simulink model "SpeedGoatLoop_v3"  (R2020b)
settings: Solver=FixedStepAuto  StartTime=0.0  StopTime=60*60*1.5  RelTol=1e-3
libraries: fl_lib x42, nesl_utility x19, SimscapeFluids_lib x4, speedgoatlib_IO132 x2, slpidlib x2
(part 1 of 2)
settings Model: SimulationMode=external  EnablePacing=on  PacingRate=100  Creator=cheap  LastModifiedBy=cheap
settings SolverCC: ConcurrentTasks=on  PositivePriorityOrder=on
settings OptimizationCC: BlockReduction=off  OptimizeBlockIOStorage=off
settings DebuggingCC: TasksWithSamePriorityMsg=none
settings HardwareCC: ProdBitPerLong=64  ProdLongLongMode=on  ProdHWDeviceType=Intel->x86-64 (Linux 64)
settings RTWCC: Description=Simulink Real-Time  SystemTargetFile=slrealtime.tlc  TemplateMakefile=slrealtime_default_tmf  Toolchain=Simulink Real-Time Toolchain  BuildConfiguration=Faster Runs  CodeExecutionProfiling=on  TargetLang=C++

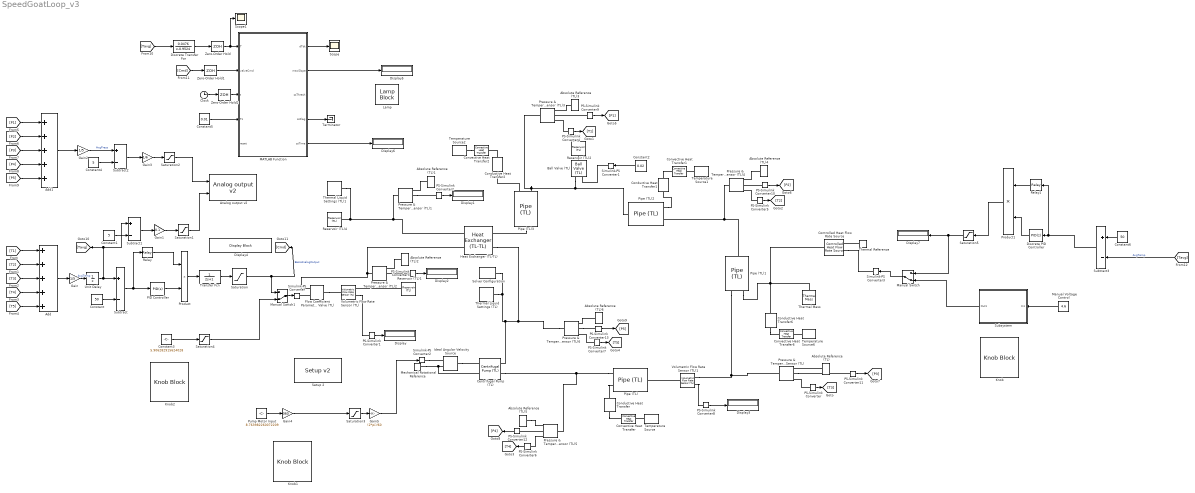
== system SpeedGoatLoop_v3 ==
  Absolute Reference (TL){,1..6} (7 alike) : fl_lib/Thermal Liquid/Elements/Absolute Reference (TL)
      settings: SourceProductBaseCode=SS
  Add : Sum  Inputs=+++++
  Add1 : Sum  Inputs=+++++
  "Analog output v2 " : speedgoatlib_IO132/Analog output v2   parModuleId=1  parSampleTime=-1  parPciSlot=-1  parDacChannels=[1 2]  parDacVoltageRange=[2 2 1 1]  parDacInitValues=[1 1]  parDacReset=[1 1]  parDacSyncOut=1  parDacDmaEnable=0  parDacActiveDmaDevices=1  parDacDmaLatency=2  parDacFrameSize=100
      settings: SourceProductName=Simulink Real-Time: Speedgoat I/O Blockset
  Ball Valve (TL) : SimscapeFluids_lib/Thermal Liquid/Valves & Orifices/Flow Control Valves/Ball Valve (TL)  valve_seat_spec=1  cone_angle=120 deg  diam_ball=1.7 in  diam_orifice=1.5 in  x_0=0 m  area_leak=1e-12 m^2  smoothing_factor=0.05  area=((1.7*pi)^2)/4 in^2  length=0.1 m  Cd=0.7  Re_c=12  mdot_A_specify=off  mdot_A_priority=None  mdot_A=1 kg/s  mdot_A_nominal_specify=off  mdot_A_nominal_unit=kg/s  mdot_A_nominal_value=1
      settings: SourceProductBaseCode=SH  InternalSimscapePortConfiguration="{\"Bottom\":[],\"Left\":[{\"id\":\"A\",\"label\":\"A\",\"type\":\"foundation.thermal_liquid.thermal_liquid\"},{\"id\":\"S\",\"label\":\"S\",\"type\":\"input\"}],\"Right\":[{\"id\":\"B\",\"label\":\"B\",\"type\":\"foundation.thermal_liquid.thermal_liquid\"}],\"Top\":[]}"
  Centrifugal Pump (TL) : SimscapeFluids_lib/Thermal Liquid/Pumps & Motors/Centrifugal Pump (TL)  pump_parameterization=1  mech_orientation=1  flow_rate_1D_TLU=[0 8.33e-5 1.67e-4 2.50e-4 3.33e-4 4.17e-4 5.00e-4 5.83e-4 6.67e-4] m^3/s  head_1D_TLU=[20 19.7 19.0 18.0 16.8 15.2 13.0 10.2 7.5] m  power_1D_TLU=[0 40 80 140 210 290 380 470 550] W  rho_ref_1D=998 kg/m^3  omega_ref_1D=363 rad/s  flow_rate_2D_TLU=[16.67, 23.33, 30, 40, 53.33, 60] lpm  omega_2D_TLU=[2450, 2800, 3150, 3500] rpm  head_2D_TLU=[25, 32.7, 42.5, 50; 24, 31.7, 41, 49; 22.7, 30.5, 39, 47.5; 20, 28, 36, 45; 15.7, 24, 32, 40; 12.5, 21, 29.5, 37.5] m  power_2D_TLU=[.28, .38, .5, .6; .31, .41, .55, .68; .33, .44, .6, .75; .36, .48, .65, .83; .38, .53, .72, .93; .39, .55, .75, .97] kW  rho_ref_2D=920 kg/m^3  omega_threshold=10 rad/s  area=((pi*2)^2)/4 in^2  mdot_A_specify=off  mdot_A_priority=None  mdot_A=1 kg/s  mdot_A_nominal_specify=off  mdot_A_nominal_unit=kg/s  mdot_A_nominal_value=1
      settings: SourceProductBaseCode=SH  InternalSimscapePortConfiguration="{\"Bottom\":[],\"Left\":[{\"id\":\"A\",\"label\":\"A\",\"type\":\"foundation.thermal_liquid.thermal_liquid\"},{\"id\":\"B\",\"label\":\"B\",\"type\":\"foundation.thermal_liquid.thermal_liquid\"}],\"Right\":[{\"id\":\"R\",\"label\":\"R\",\"type\":\"foundation.mechanical.rotational.rotational\"},{\"id\":\"C\",\"label\":\"C\",\"type\":\"foundation.mechanical.rotational.rotational\"}],\"Top\":[]}"
  Clock : Clock
  Conductive Heat Transfer{,1..2,6} (4 alike) : fl_lib/Thermal/Thermal Elements/Conductive Heat Transfer  area=1e-4 m^2  thickness=0.1 m  th_cond=16.2 W/(K*m)  T_specify=off  T_priority=None  T=0 K  T_nominal_specify=off  T_nominal_unit=K  T_nominal_value=1  Q_specify=off  Q_priority=None  Q=0 W  Q_nominal_specify=off  Q_nominal_unit=W  Q_nominal_value=1
  Constant : Constant  Value=50
  Constant1 : Constant  Value=5
  Constant2 : Constant  Value=0.02
  Constant3 : Constant  Value=5.906282915624028
  Constant4 : Constant  Value=5
  Constant5 : Constant  Value=0.01
  Constant6 : Constant  Value=50
  Controlled Heat Flow Rate Source : fl_lib/Thermal/Thermal Sources/Controlled Heat Flow Rate Source
  Convective Heat Transfer : fl_lib/Thermal/Thermal Elements/Convective Heat Transfer  area=pi*50*(656.10+50.8+179.35+254) mm^2  heat_tr_coeff=10 W/(K*m^2)  T_specify=off  T_priority=None  T=0 K  T_nominal_specify=off  T_nominal_unit=K  T_nominal_value=1  Q_specify=off  Q_priority=None  Q=0 W  Q_nominal_specify=off  Q_nominal_unit=W  Q_nominal_value=1
  Convective Heat Transfer1 : fl_lib/Thermal/Thermal Elements/Convective Heat Transfer  area=pi*50*(656.10+50.8+179.35+254) mm^2  heat_tr_coeff=10 W/(K*m^2)  T_specify=off  T_priority=None  T=0 K  T_nominal_specify=off  T_nominal_unit=K  T_nominal_value=1  Q_specify=off  Q_priority=None  Q=0 W  Q_nominal_specify=off  Q_nominal_unit=W  Q_nominal_value=1
  Convective Heat Transfer2 : fl_lib/Thermal/Thermal Elements/Convective Heat Transfer  area=pi*50*(656.10+50.8+179.35+254) mm^2  heat_tr_coeff=10 W/(K*m^2)  T_specify=off  T_priority=None  T=0 K  T_nominal_specify=off  T_nominal_unit=K  T_nominal_value=1  Q_specify=off  Q_priority=None  Q=0 W  Q_nominal_specify=off  Q_nominal_unit=W  Q_nominal_value=1
  Convective Heat Transfer6 : fl_lib/Thermal/Thermal Elements/Convective Heat Transfer  area=pi*50*(6000) mm^2  heat_tr_coeff=10 W/(K*m^2)  T_specify=off  T_priority=None  T=0 K  T_nominal_specify=off  T_nominal_unit=K  T_nominal_value=1  Q_specify=off  Q_priority=None  Q=0 W  Q_nominal_specify=off  Q_nominal_unit=W  Q_nominal_value=1
  Discrete Transfer Fcn : DiscreteTransferFcn  Numerator=[0.0476]  Denominator=[1 -0.9524]  SampleTime=0.01
  Discrete PID Controller : slpidlib/PID Controller  Controller=PID  Form=Parallel  TimeDomain=Discrete-time  UseExternalTs=off  SampleTime=0.01  IntegratorMethod=Forward Euler  FilterMethod=Forward Euler  ControllerParametersSource=internal  P=100  I=1.5  D=0  UseFilter=on  N=100  TunerSelectOption=Transfer Function Based (PID Tuner App)  InitialConditionSource=internal  InitialConditionForIntegrator=0  InitialConditionForFilter=0  DifferentiatorICPrevScaledInput=0  ExternalReset=none  TrackingMode=off  Kt=1  LimitOutput=on  SatLimitsSource=internal  UpperSaturationLimit=10000  LowerSaturationLimit=0  LinearizeAsGain=off  AntiWindupMode=back-calculation  Kb=1  POutMin=[]  POutMax=[]  IOutMin=[]  IOutMax=[]  DOutMin=[]  DOutMax=[]  NOutMin=[]  NOutMax=[]  SumOutMin=[]  SumOutMax=[]  SaturationOutMin=[]  SaturationOutMax=[]  PParamMin=[]  PParamMax=[]  IParamMin=[]  IParamMax=[]  DParamMin=[]  DParamMax=[]  NParamMin=[]  NParamMax=[]  KbParamMin=[]  KbParamMax=[]  KtParamMin=[]  KtParamMax=[]  KbOutMin=[]  KbOutMax=[]  KtOutMin=[]  KtOutMax=[]  IntegratorOutMin=[]  IntegratorOutMax=[]  FilterOutMin=[]  FilterOutMax=[]  SumI1OutMin=[]  SumI1OutMax=[]  SumI2OutMin=[]  SumI2OutMax=[]  SumI3OutMin=[]  SumI3OutMax=[]  SumI4OutMin=[]  SumI4OutMax=[]  SumDOutMin=[]  SumDOutMax=[]  DifferentiatorOutMin=[]  DifferentiatorOutMax=[]  FilterDiffOutCoefMin=[]  FilterDiffOutCoefMax=[]  ReciprocalOutMin=[]  ReciprocalOutMax=[]  SumDenOutMin=[]  SumDenOutMax=[]  SumNumOutMin=[]  SumNumOutMax=[]  DivideOutMin=[]  DivideOutMax=[]  UdiffTsProdOutMin=[]  UdiffTsProdOutMax=[]  NTsProdOutMin=[]  NTsProdOutMax=[]  UintegralTsProdOutMin=[]  UintegralTsProdOutMax=[]  UngainTsProdOutMin=[]  UngainTsProdOutMax=[]  IntegratorContinuousStateAttributes=''  IntegratorStateMustResolveToSignalObject=off  IntegratorRTWStateStorageClass=Auto  FilterContinuousStateAttributes=''  FilterStateMustResolveToSignalObject=off  FilterRTWStateStorageClass=Auto  ParallelPVariant=InternalParameters  IdealPVariant=Disabled  IVariant=InternalParameters  DVariant=InternalParameters  IntegratorVariant=Discrete  SatVariant=Enabled  AWVariant=BackCalculation  PCopyVariant=Disabled  TRVariant=Disabled  FdbkBlocksVariant=Forward  IdealPFdbkVariant=Disabled  SatFdbkVariant=Disabled  DerivativeFilterVariant=ForwardEulerFilter  NVariant=InternalParameters  NCopyVariant=Disabled  FilterICVariant=InternalICsFilter  IntegratorICVariant=InternalICs  ExternalResetVariant=Disabled  TRSumVariant=Passthrough  SumFdbkVariant=Disabled  SumVariant=Sum_PID  TsampFilterVariant=InternalTs  TsampNgainVariant=Passthrough  TsampIntegralVariant=Passthrough  ExternalSaturationOutDataTypeStr=Inherit: Same as second input
  Display{,1..3,5..7} (7 alike) : Display
  Display4 : DisplayBlock  LabelPosition=Hide  Format=short  Transparency=1
  Flow Coefficient Parameterized Valve (TL) : SimscapeFluids_lib/Thermal Liquid/Valves & Orifices/Flow Coefficient Parameterized Valve (TL)  flow_coeff_spec=fluids.thermal_liquid.valves.enum.flow_coeff_spec.cv  Cv_max=1  Cv_min=1e-4  Kv_max=1  Kv_min=1e-4  valve_character=fluids.thermal_liquid.valves.enum.valve_opening_spec.linear  rangeability=50  alpha=2  area=((0.75*pi)^2)/4 in^2  length=3 in  Re_c=12  smoothing_factor=0.02  opening_dynamic=simscape.enum.onoff.off  tau=0.1 s  mdot_A_specify=off  mdot_A_priority=None  mdot_A=1 kg/s  mdot_A_nominal_specify=off  mdot_A_nominal_unit=kg/s  mdot_A_nominal_value=1  area_dynamic_specify=off  area_dynamic_priority=High  area_dynamic=1e-10 m^2  area_dynamic_nominal_specify=off  area_dynamic_nominal_unit=m^2  area_dynamic_nominal_value=1
      settings: SourceProductBaseCode=SH  InternalSimscapePortConfiguration="{\"Bottom\":[],\"Left\":[{\"id\":\"A\",\"label\":\"A\",\"type\":\"foundation.thermal_liquid.thermal_liquid\"},{\"id\":\"L\",\"label\":\"L\",\"type\":\"input\"}],\"Right\":[{\"id\":\"B\",\"label\":\"B\",\"type\":\"foundation.thermal_liquid.thermal_liquid\"}],\"Top\":[]}"
  Gain : Gain  Gain=1/5
  Gain1 : Gain  Gain=0.1
  Gain2 : Gain  Gain=1/5
  Gain3 : Gain  Gain=1/6
  Gain4 : Gain  Gain=360
  Gain5 : Gain  Gain=(2*pi)/60
  Heat Exchanger (TL-TL) : SimscapeFluids_lib/Fluid Network Interfaces/Heat Exchangers/Heat Exchanger (TL-TL)  hex_type=fluids.interfaces.enum.flow_arrangement_spec.shell_tube  cross_type=fluids.interfaces.enum.cross_flow_heat_exchanger_TL_TL_spec.mixed_mixed  shell_num=1  NTU_TLU=[.5, 1, 2, 3, 4, 5]  CR_TLU=[0, .25, .5, .75, 1]  eff_TLU=[.3, .3, .3, .3, .3; .6, .55, .5, .47, .43; .85, .76, .68, .61, .55; .94, .83, .72, .65, .58; .98, .86, .75, .66, .58; .99, .86, .75, .66, .58]  wall_thermal_dynamics=simscape.enum.onoff.on  thermal_mass_wall=447 J/K  R_wall=1.984E-3 K/W  min_flow_area_1=1.16E-3 m^2  Dh_press_1=0.00451 m  liquid_volume_1=3E-3 m^3  Re_lam_1=2000  Re_tur_1=4000  pressure_loss_spec_1=fluids.interfaces.enum.pressure_loss_spec.constant  min_flow_area_2=9.19E-4 m^2  Dh_press_2=0.004572 m  liquid_volume_2=8.41E-4 m^3  Re_lam_2=2000  Re_tur_2=4000  pressure_loss_spec_2=fluids.interfaces.enum.pressure_loss_spec.tube_correlation  pressure_loss_coeff_1=0.1  length_press_1=1 m  length_add_1=0.1 m  roughness_1=15e-6 m  Re_friction_TLU_1=[400, 1000, 1500, 3000, 4000, 6000, 10000, 20000, 40000, 60000, 100000, 100000000]  friction_factor_TLU_1=[.264, .112, .071, .0417, .0387, .0268, .025, .0232, .0226, .022, .0214, .0214]  shape_factor_1=64  Re_Euler_TLU_1=[50, 500, 1000, 2000]  Euler_TLU_1=[4.4505, .6864, .4791, .3755]  pressure_loss_coeff_2=0.1  length_press_2=0.9144 m  length_add_2=0.4 m  roughness_2=15e-6 m  Re_friction_TLU_2=[400, 1000, 1500, 3000, 4000, 6000, 10000, 20000, 40000, 60000, 100000, 100000000]  friction_factor_TLU_2=[.264, .112, .071, .0417, .0387, .0268, .025, .0232, .0226, .022, .0214, .0214]  shape_factor_2=64  Re_Euler_TLU_2=[50, 500, 1000, 2000]  Euler_TLU_2=[4.4505, .6864, .4791, .3755]  heat_transfer_spec_1=fluids.interfaces.enum.heat_transfer_spec.constant  heat_transfer_spec_2=fluids.interfaces.enum.heat_transfer_spec.tube_correlation  heat_coeff_1=100 W/(m^2 * K)  length_heat_1=1 m  Nu_lam_1=3.66  Re_Colburn_TLU_1=[100, 150, 1000]  Colburn_factor_TLU_1=[.019, .013, .002]  Re_Nu_TLU_1=[100, 150, 1000]  Pr_Nu_TLU_1=[1, 10]  Nu_TLU_1=[3.72, 4.21; 3.75, 4.44; 4.21, 7.15]  heat_coeff_2=100 W/(m^2 * K)  length_heat_2=0.9144 m  Nu_lam_2=3.66  Re_Colburn_TLU_2=[100, 150, 1000]  Colburn_factor_TLU_2=[.019, .013, .002]  Re_Nu_TLU_2=[100, 150, 1000]  Pr_Nu_TLU_2=[1, 10]  Nu_TLU_2=[3.72, 4.21; 3.75, 4.44; 4.21, 7.15]  heat_transfer_area_1=1.022 m^2  fouling_factor_1=1e-4 m^2*K/W  min_heat_coeff_1=3000 W/(m^2 * K)  heat_transfer_area_2=0.735 m^2  fouling_factor_2=1e-4 m^2*K/W  min_heat_coeff_2=10000 W/(m^2 * K)  dynamic_compressibility_1=simscape.enum.onoff.on  T0_1=10 degC  p0_1=0.101325 MPa  dynamic_compressibility_2=simscape.enum.onoff.on  T0_2=24 degC  p0_2=0.101325 MPa  mdot1_TLU=[.3, .5, .6, .7, 1, 1.4, 1.9, 2.3] kg/s  mdot2_TLU=[.3, .5, 1, 1.3, 1.7, 2, 2.6, 3.3] kg/s  SD_TLU=[.324, .3533, .404, .4253, .4333, .4373, .4453, .4533; .3813, .424, .496, .5307, .544, .5547, .5693, .5787; .4267, .4827, .5813, .6173, .6413, .6573, .672, .6827; .4613, .528, .64, .6987, .7267, .7467, .7707, .7853; .5533, .6467, .8227, .928, .9853, 1.0187, 1.0653, 1.0973; .58, .688, .8853, 1.0147, 1.08, 1.124, 1.176, 1.2147; .624, .7467, .992, 1.148, 1.244, 1.304, 1.3773, 1.4267; .656, .7907, 1.0667, 1.26, 1.376, 1.452, 1.548, 1.612] kW/K  Q_check=fluids.interfaces.enum.SD_max_check.warning  mdot_dp_TLU_1=[.3, .5, 1, 1.5, 2, 2.5] kg/s  p_diff_TLU_1=[3, 5, 10, 25, 35, 50] * 1e-3 MPa  T_ref_in_1=293.15 K  p_ref_in_1=0.101325 MPa  mdot_threshold_1=1e-3 kg/s  area_1=0.01 m^2  mdot_dp_TLU_2=[.3, .5, 1, 1.5, 2, 2.5] kg/s  p_diff_TLU_2=[3, 5, 10, 25, 35, 50] * 1e-3 MPa  T_ref_in_2=293.15 K  p_ref_in_2=0.101325 MPa  mdot_threshold_2=1e-3 kg/s  area_2=0.01 m^2
      settings: SourceProductBaseCode=SH  InternalSimscapePortConfiguration="{\"Bottom\":[],\"Left\":[{\"id\":\"A1\",\"label\":\"A1\",\"type\":\"foundation.thermal_liquid.thermal_liquid\"},{\"id\":\"B1\",\"label\":\"B1\",\"type\":\"foundation.thermal_liquid.thermal_liquid\"}],\"Right\":[{\"id\":\"A2\",\"label\":\"A2\",\"type\":\"foundation.thermal_liquid.thermal_liquid\"},{\"id\":\"B2\",\"label\":\"B2\",\"type\":\"foundation.thermal_liquid.thermal_liquid\"}],\"Top\":[]}"
  Ideal Angular Velocity Source : fl_lib/Mechanical/Mechanical Sources/Ideal Angular Velocity Source
  Knob : KnobBlock  ScaleMax=20
  Knob1 : KnobBlock  ScaleMax=10
  Knob2 : KnobBlock  ScaleMax=1
  Lamp : LampBlock
  MATLAB Function : MATLAB Function  TreatAsAtomicUnit=on
  Manual Switch : ManualSwitch  CurrentSetting=0
  Manual Switch1 : ManualSwitch  CurrentSetting=0
  Manual Voltage Control : Constant  Value=4.6
  Mechanical Rotational Reference : fl_lib/Mechanical/Rotational Elements/Mechanical Rotational Reference
  PID Controller : slpidlib/PID Controller  Controller=PID  Form=Parallel  TimeDomain=Continuous-time  UseExternalTs=off  SampleTime=-1  IntegratorMethod=Forward Euler  FilterMethod=Forward Euler  ControllerParametersSource=internal  P=0.1  I=1e-5  D=0  UseFilter=on  N=100  TunerSelectOption=Transfer Function Based (PID Tuner App)  InitialConditionSource=internal  InitialConditionForIntegrator=0  InitialConditionForFilter=0  DifferentiatorICPrevScaledInput=0  ExternalReset=none  TrackingMode=off  Kt=1  LimitOutput=on  SatLimitsSource=internal  UpperSaturationLimit=1  LowerSaturationLimit=0  LinearizeAsGain=on  AntiWindupMode=clamping  Kb=1  POutMin=[]  POutMax=[]  IOutMin=[]  IOutMax=[]  DOutMin=[]  DOutMax=[]  NOutMin=[]  NOutMax=[]  SumOutMin=[]  SumOutMax=[]  SaturationOutMin=[]  SaturationOutMax=[]  PParamMin=[]  PParamMax=[]  IParamMin=[]  IParamMax=[]  DParamMin=[]  DParamMax=[]  NParamMin=[]  NParamMax=[]  KbParamMin=[]  KbParamMax=[]  KtParamMin=[]  KtParamMax=[]  KbOutMin=[]  KbOutMax=[]  KtOutMin=[]  KtOutMax=[]  IntegratorOutMin=[]  IntegratorOutMax=[]  FilterOutMin=[]  FilterOutMax=[]  SumI1OutMin=[]  SumI1OutMax=[]  SumI2OutMin=[]  SumI2OutMax=[]  SumI3OutMin=[]  SumI3OutMax=[]  SumI4OutMin=[]  SumI4OutMax=[]  SumDOutMin=[]  SumDOutMax=[]  DifferentiatorOutMin=[]  DifferentiatorOutMax=[]  FilterDiffOutCoefMin=[]  FilterDiffOutCoefMax=[]  ReciprocalOutMin=[]  ReciprocalOutMax=[]  SumDenOutMin=[]  SumDenOutMax=[]  SumNumOutMin=[]  SumNumOutMax=[]  DivideOutMin=[]  DivideOutMax=[]  UdiffTsProdOutMin=[]  UdiffTsProdOutMax=[]  NTsProdOutMin=[]  NTsProdOutMax=[]  UintegralTsProdOutMin=[]  UintegralTsProdOutMax=[]  UngainTsProdOutMin=[]  UngainTsProdOutMax=[]  IntegratorContinuousStateAttributes=''  IntegratorStateMustResolveToSignalObject=off  IntegratorRTWStateStorageClass=Auto  FilterContinuousStateAttributes=''  FilterStateMustResolveToSignalObject=off  FilterRTWStateStorageClass=Auto  ParallelPVariant=InternalParameters  IdealPVariant=Disabled  IVariant=InternalParameters  DVariant=InternalParameters  IntegratorVariant=Continuous  SatVariant=Enabled  AWVariant=ContClampingParallel  PCopyVariant=Disabled  TRVariant=Disabled  FdbkBlocksVariant=Forward  IdealPFdbkVariant=Disabled  SatFdbkVariant=Disabled  DerivativeFilterVariant=ContFilter  NVariant=InternalParameters  NCopyVariant=Disabled  FilterICVariant=InternalICsFilter  IntegratorICVariant=InternalICs  ExternalResetVariant=Disabled  TRSumVariant=Passthrough  SumFdbkVariant=Disabled  SumVariant=Sum_PID  TsampFilterVariant=InternalTs  TsampNgainVariant=Passthrough  TsampIntegralVariant=Passthrough  ExternalSaturationOutDataTypeStr=Inherit: Same as second input
  PS-Simulink Converter{,4..7} (5 alike) : nesl_utility/PS-Simulink Converter  PhysicalDomain=network_engine_domain  SubClassName=ps_output  LeftPortType=input  RightPortType=output  PseudoPeriodic=off  Frequencies=[]  Unit=degC  AffineConversion=on
  PS-Simulink Converter1 : nesl_utility/PS-Simulink Converter  PhysicalDomain=network_engine_domain  SubClassName=ps_output  LeftPortType=input  RightPortType=output  PseudoPeriodic=off  Frequencies=[]  Unit=gpm  AffineConversion=on
  PS-Simulink Converter{2,9..13} (6 alike) : nesl_utility/PS-Simulink Converter  PhysicalDomain=network_engine_domain  SubClassName=ps_output  LeftPortType=input  RightPortType=output  PseudoPeriodic=off  Frequencies=[]  Unit=psi  AffineConversion=on
  PS-Simulink Converter3 : nesl_utility/PS-Simulink Converter  PhysicalDomain=network_engine_domain  SubClassName=ps_output  LeftPortType=input  RightPortType=output  PseudoPeriodic=off  Frequencies=[]  Unit=inherit  AffineConversion=off
  PS-Simulink Converter8 : nesl_utility/PS-Simulink Converter  PhysicalDomain=network_engine_domain  SubClassName=ps_output  LeftPortType=input  RightPortType=output  PseudoPeriodic=off  Frequencies=[]  Unit=gpm  AffineConversion=on
  Pipe (TL) : fl_lib/Thermal Liquid/Elements/Pipe (TL)  length=572+698.5+113+656.1+50.8+179.35+254 mm  area=((1.7*pi)^2)/4 in^2  Dh=1.5 in  length_add=1 m  roughness=15e-6 m  Re_lam=2000  Re_tur=4000  shape_factor=64  Nu_lam=3.66  dynamic_compressibility=simscape.enum.onoff.on  inertia=simscape.enum.onoff.off  p0=40 psi  T0=24 degC  mdot0=0 kg/s
      settings: SourceProductBaseCode=SS
  Pipe (TL)1 : fl_lib/Thermal Liquid/Elements/Pipe (TL)  length=1666.08+113 mm  area=((50*pi)^2)/4 mm^2  Dh=1.5 in  length_add=1 m  roughness=15e-6 m  Re_lam=2000  Re_tur=4000  shape_factor=64  Nu_lam=3.66  dynamic_compressibility=simscape.enum.onoff.on  inertia=simscape.enum.onoff.off  p0=0.12 MPa  T0=24 degC  mdot0=0 kg/s
      settings: SourceProductBaseCode=SS
  Pipe (TL)2 : fl_lib/Thermal Liquid/Elements/Pipe (TL)  length=322.66+283.65+665.16+113+331.45+863.6 mm  area=((1.7*pi)^2)/4 in^2  Dh=1.5 in  length_add=1 m  roughness=15e-6 m  Re_lam=2000  Re_tur=4000  shape_factor=64  Nu_lam=3.66  dynamic_compressibility=simscape.enum.onoff.on  inertia=simscape.enum.onoff.off  p0=0.101325 MPa  T0=24 degC  mdot0=0 kg/s
      settings: SourceProductBaseCode=SS
  Pipe (TL)3 : fl_lib/Thermal Liquid/Elements/Pipe (TL)  length=211.02+1024.8+164.52+317.72 mm  area=((1.7*pi)^2)/4 in^2  Dh=1.5 in  length_add=1 m  roughness=15e-6 m  Re_lam=2000  Re_tur=4000  shape_factor=64  Nu_lam=3.66  dynamic_compressibility=simscape.enum.onoff.on  inertia=simscape.enum.onoff.off  p0=0.101325 MPa  T0=24 degC  mdot0=0 kg/s
      settings: SourceProductBaseCode=SS
  Pressure & Temperature Sensor (TL){,1..6} (7 alike) : fl_lib/Thermal Liquid/Sensors/Pressure & Temperature Sensor (TL)
      settings: SourceProductBaseCode=SS  InternalSimscapePortConfiguration="{\"Bottom\":[],\"Left\":[{\"id\":\"A\",\"label\":\"A\",\"type\":\"foundation.thermal_liquid.thermal_liquid\"}],\"Right\":[{\"id\":\"B\",\"label\":\"B\",\"type\":\"foundation.thermal_liquid.thermal_liquid\"},{\"id\":\"P\",\"label\":\"P\",\"type\":\"output\"},{\"id\":\"T\",\"label\":\"T\",\"type\":\"output\"}],\"Top\":[]}"
  Product : Product
  Product1 : Product
  Pump Motor Input : Constant  Value=8.763982260072209
  Relay : Relay  OnSwitchValue=48  OffSwitchValue=46
  Relay1 : Relay  OnSwitchValue=48  OffSwitchValue=46  OnOutputValue=0  OffOutputValue=1
  Reservoir (TL)1 : fl_lib/Thermal Liquid/Elements/Reservoir (TL)  pressure_spec=foundation.enum.pressure_spec.atmospheric  reservoir_pressure=0.101325 MPa  reservoir_temperature=10 degC  area=((pi*1.5)^2)/4 in^2
      settings: SourceProductBaseCode=SS
  Reservoir (TL)2 : fl_lib/Thermal Liquid/Elements/Reservoir (TL)  pressure_spec=foundation.enum.pressure_spec.atmospheric  reservoir_pressure=0.101325 MPa  reservoir_temperature=15 degC  area=((pi*1.5)^2)/4 in^2
      settings: SourceProductBaseCode=SS
  Reservoir (TL)4 : fl_lib/Thermal Liquid/Elements/Reservoir (TL)  pressure_spec=foundation.enum.pressure_spec.specified  reservoir_pressure=60 psi  reservoir_temperature=10 degC  area=((pi*1.5)^2)/4 in^2
      settings: SourceProductBaseCode=SS
  Saturation : Saturate  UpperLimit=0.98  LowerLimit=0.0002
  Saturation1 : Saturate  UpperLimit=10  LowerLimit=0
  Saturation2 : Saturate  UpperLimit=90  LowerLimit=20
  Saturation3 : Saturate  UpperLimit=3600  LowerLimit=0
  Saturation4 : Saturate  LowerLimit=7e-5
  Saturation5 : Saturate  UpperLimit=10000  LowerLimit=0
  Scope : Scope
  Scope1 : Scope
  "Setup 2 " : speedgoatlib_IO132/Setup v2   parPciSlot=-1  parModuleId=1  parInterModuleSync=None  parConvClockBaseRate=20MHz  parConvClock1Divider=20000  parConvClock2Divider=20000  parFrameTriggerEnable=off  parFrameTriggerDivider=10  parConvClock1BaseRate=1  parConvClock2BaseRate=1  parFrameTriggerClock=1  parAdcChannels=[1]  parAdcRange1=+-10V  parAdcOversampling1=None  parAdcAutoCorrection=on  parAdcContSampling=off  parAdcVoltageRange=2  parAdcOversamplRate=1  parAdcDmaEnable=off  parAdcDmaClock=Clock 1  parAdcFrameSize_=100  parAdcSampleTime_=-1  parAdcActiveDmaDevices=[1]  parAdcFrameTriggerEnable=0  parAdcFrameSize=100  parAdcSampleTime=0.1  parDacChannels=[1 2]  parDacInitValues=1  parDacReset=1  parDacRange1=0-10V  parDacRange2=0-10V  parDacRange3=0-5V  parDacRange4=0-5V  parDacVoltageRange=[2 2 1 1]  parDacAutoCorrection=on  parDacSyncOut=on  parDacDmaEnable=off  parDacDmaLatency=Until next frame  parDacDmaClock=Clock 1  parDacFrameSize_=100  parDacSampleTime_=-1  parDacActiveDmaDevices=[1]  parDacFrameTriggerEnable=0  parDacFrameSize=100  parDacSampleTime=0.1  parDoChannels=[1 2]  parDoInitValues=0  parDoReset=1  parDiChannels=[3 4]  parDiDebounceEnable=off  parDiDebounceTime=0  parDiDebounceValue=0  parDioPullRefFront=Pull-up 3.3V  parDioPullRefRear=Floating
      settings: SourceProductName=Simulink Real-Time: Speedgoat Library
  Simulink-PS Converter{,1..3} (4 alike) : nesl_utility/Simulink-PS Converter  PhysicalDomain=network_engine_domain  SubClassName=ps_input  LeftPortType=input  RightPortType=output  PseudoPeriodic=off  Frequencies=[]  NoiseDistribution=none  NoiseParameters=[]  Unit=1  AffineConversion=off  FilteringAndDerivatives=provide  SimscapeFilterOrder=1  InputFilterTimeConstant=0.001  UdotUserProvided=0
  Solver Configuration : nesl_utility/Solver Configuration  PhysicalDomain=network_engine_domain  SubClassName=solver  LeftPortType=input  RightPortType=generic  Tones=[]  Harmonics=[]  SimulateNoise=off  Profile=off  UseLocalSampling=off  EnableSwitchedLinearOptims=on  FrequencyDomain=off  UseCCode=off  RelTol=0.001  AbsTol=1e-06  MinStep=1e-09  ToWorkspace=off  RevertToSquareIcSolve=off  NumHomotopyIterations=100  PhasorMode=off  PhasorModeNumHarmonics=1  DoDC=off  ResidualTolerance=1e-09  UseLocalSolver=on  LocalSolverChoice=NE_BACKWARD_EULER_ADVANCER  LocalSolverSampleTime=0.01  DoFixedCost=on  MaxNonlinIter=3  MaxModeIter=2  ComputeImpulses=off  ImpulseIterations=2  LinearAlgebra=auto  EquationFormulation=NE_TIME_EF  DelaysMemoryBudget=1024  AutomaticFiltering=on  FilteringTimeConstant=0.001  PartitionStorageMethod=AS_NEEDED  PartitionMemoryBudget=1024  PartitionMethod=ROBUST
  Subsystem : Subsystem
      settings: PortSchema="{\"entries\":[{\"content\":{\"sides\":[{\"content\":{\"connectorIds\":[\"Out1\"]},\"type\":\"ConnectorPlacement.EquallySpacedRectSide\",\"uuid\":\"fb919825-1b2f-4c31-9805-0967e26cfa90\"},{\"content\":{\"connectorIds\":[\"In1\"],\"side\":\"RIGHT\"},\"type\":\"ConnectorPlacement.EquallySpacedRectSide\",\"uuid\":\"9136b45b-edcb-43b5-a0c1-cf6d919585f5\"},{\"content\":{\"connectorIds\":[],\"side\":\"TOP\"},\"type\":\"ConnectorPlacement.EquallySpacedRectSide\",\"uuid\":\"eaf0a6cf-ad87-41c1-a56b-7e33ba526407\"}]},\"type\":\"ConnectorPlacement.EquallySpacedConnector\",\"uuid\":\"77377397-7f65-431b-b464-9c22985d1642\"}],\"packageUris\":[\"http://schema.mathworks.com/mf0/Connector/R2020b\"],\"version\":\"1.0\"}"
  Subtract{,1..3} (4 alike) : Sum  Inputs=+-
  Temperature Source{,1..2,6} (4 alike) : fl_lib/Thermal/Thermal Sources/Temperature Source  temperature=293.15 K
  Terminator : Terminator
  Thermal Liquid Settings (TL) : fl_lib/Thermal Liquid/Utilities/Thermal Liquid Settings (TL)  table_dimensions=foundation.enum.table_dimensions_TL.two_dimensional  T_TLU=[5 : 10 : 105]' degC  p_TLU=[0.01, 0.1, 5 : 5 : 50] MPa  p_atm=0.101325 MPa  pT_region_flag=foundation.enum.pT_region_TL.min_max  T_min=5 degC  T_max=105 degC  p_min=0.05 MPa  p_max=50 MPa  T_min_1D=273.16 K  T_max_1D=363.16 K  p_min_1D=0.05 MPa  p_max_1D=50 MPa  pT_validity_TLU=[1, 1, 1, 1, 1, 1, 1, 1, 1, 1, 1, 1; 1, 1, 1, 1, 1, 1, 1, 1, 1, 1, 1, 1; 1, 1, 1, 1, 1, 1, 1, 1, 1, 1, 1, 1; 1, 1, 1, 1, 1, 1, 1, 1, 1, 1, 1, 1; 1, 1, 1, 1, 1, 1, 1, 1, 1, 1, 1, 1; 0, 1, 1, 1, 1, 1, 1, 1, 1, 1, 1, 1; 0, 1, 1, 1, 1, 1, 1, 1, 1, 1, 1, 1; 0, 1, 1, 1, 1, 1, 1, 1, 1, 1, 1, 1; 0, 1, 1, 1, 1, 1, 1, 1, 1, 1, 1, 1; 0, 1, 1, 1, 1, 1, 1, 1, 1, 1, 1, 1; 0, 0, 1, 1, 1, 1, 1, 1, 1, 1, 1, 1]  rho_parameterization_2D=foundation.enum.rho_parameterization_2D.rho_beta_alpha  rho_parameterization_1D=foundation.enum.rho_parameterization_1D.rho_vector  rho_TLU=[999.7973, 999.8431, 1002.3216, 1004.8218, 1007.293, 1009.7358, 1012.1506, 1014.5379, 1016.8979, 1019.2311, 1021.538, 1023.8188; 999.6579, 999.7009, 1002.0303, 1004.382, 1006.7084, 1009.0101, 1011.2874, 1013.5407, 1015.7703, 1017.9766, 1020.1599, 1022.3206; 998.1632, 998.2045, 1000.4375, 1002.6924, 1004.9239, 1007.1324, 1009.3183, 1011.4819, 1013.6236, 1015.7438, 1017.8428, 1019.921; 995.6057, 995.6458, 997.81864, 1000.0128, 1002.1841, 1004.3332, 1006.4603, 1008.566, 1010.6505, 1012.7144, 1014.758, 1016.7815; 992.1724, 992.2119, 994.35133, 996.5113, 998.6484, 1000.7633, 1002.8563, 1004.928, 1006.9788, 1009.009, 1011.0192, 1013.0097; 988.02, 988.0299, 990.15684, 992.3035, 994.4268, 996.5273, 998.6056, 1000.6622, 1002.6976, 1004.7123, 1006.7067, 1008.6813; 983.18, 983.1901, 985.3217, 987.4721, 989.5983, 991.7008, 993.7803, 995.8374, 997.8726, 999.8864, 1001.8795, 1003.8522; 977.75, 977.7583, 979.9094, 982.0783, 984.2216, 986.34, 988.4343, 990.505, 992.5529, 994.5786, 996.5825, 998.5654; 971.77, 971.7836, 973.96734, 976.1678, 978.3409, 980.4876, 982.6087, 984.7049, 986.7768, 988.8254, 990.8511, 992.8545; 965.26, 965.3023, 967.53107, 969.7753, 971.9901, 974.1764, 976.3354, 978.4676, 980.5741, 982.6556, 984.7129, 986.7465; 958.62, 958.6315, 960.627, 962.9267, 965.1944, 967.4314, 969.6387, 971.8173, 973.9681, 976.0921, 978.19, 980.2628] kg/m^3  beta_TLU=[1.9649, 1.9654, 1.9929, 2.0213, 2.0499, 2.0787, 2.1078, 2.1372, 2.1668, 2.1966, 2.2268, 2.2572; 2.0913, 2.0918, 2.1191, 2.1471, 2.1752, 2.2036, 2.2322, 2.261, 2.2899, 2.3191, 2.3485, 2.3781; 2.1786, 2.1791, 2.2067, 2.235, 2.2634, 2.2919, 2.3206, 2.3494, 2.3784, 2.4075, 2.4367, 2.4661; 2.2332, 2.2337, 2.2619, 2.2908, 2.3197, 2.3487, 2.3778, 2.407, 2.4363, 2.4657, 2.4951, 2.5246; 2.26, 2.2605, 2.2895, 2.3191, 2.3487, 2.3784, 2.4081, 2.4378, 2.4675, 2.4973, 2.5272, 2.5571; 2.2638, 2.2638, 2.2936, 2.324, 2.3544, 2.3848, 2.4151, 2.4455, 2.4758, 2.5062, 2.5365, 2.5669; 2.2472, 2.2472, 2.2779, 2.3092, 2.3403, 2.3715, 2.4025, 2.4336, 2.4646, 2.4955, 2.5264, 2.5573; 2.214, 2.214, 2.2455, 2.2776, 2.3096, 2.3415, 2.3733, 2.405, 2.4367, 2.4683, 2.4998, 2.5313; 2.1668, 2.1668, 2.1992, 2.2321, 2.2649, 2.2976, 2.3301, 2.3626, 2.3949, 2.4272, 2.4593, 2.4914; 2.1081, 2.1081, 2.1413, 2.175, 2.2086, 2.2421, 2.2754, 2.3085, 2.3415, 2.3744, 2.4072, 2.4399; 2.0494, 2.0494, 2.0739, 2.1084, 2.1428, 2.177, 2.211, 2.2449, 2.2786, 2.3121, 2.3455, 2.3788] GPa  alpha_TLU=1e-4 * [-.679, -.676, -.49, -.307, -.13, .041, .206, .365, .519, .668, .811, .949; .878, .881, .998, 1.114, 1.227, 1.337, 1.445, 1.549, 1.651, 1.75, 1.846, 1.939; 2.068, 2.069, 2.141, 2.213, 2.283, 2.352, 2.42, 2.486, 2.551, 2.614, 2.676, 2.736; 3.034, 3.035, 3.074, 3.113, 3.152, 3.191, 3.229, 3.267, 3.305, 3.341, 3.377, 3.413; 3.855, 3.856, 3.87, 3.884, 3.899, 3.914, 3.93, 3.946, 3.961, 3.977, 3.993, 4.009; 4.578, 4.578, 4.572, 4.566, 4.562, 4.558, 4.555, 4.552, 4.55, 4.549, 4.548, 4.547; 5.233, 5.233, 5.209, 5.186, 5.165, 5.144, 5.125, 5.107, 5.09, 5.074, 5.059, 5.045; 5.84, 5.84, 5.801, 5.762, 5.725, 5.691, 5.657, 5.625, 5.595, 5.566, 5.538, 5.512; 6.414, 6.414, 6.36, 6.307, 6.256, 6.208, 6.161, 6.117, 6.074, 6.033, 5.994, 5.956; 6.967, 6.967, 6.898, 6.831, 6.766, 6.705, 6.646, 6.589, 6.535, 6.482, 6.432, 6.384; 7.519, 7.519, 7.423, 7.342, 7.264, 7.189, 7.118, 7.049, 6.983, 6.92, 6.859, 6.8] 1/K  rho_TLU_2=[999.7973, 999.8431, 1002.3216, 1004.8218, 1007.293, 1009.7358, 1012.1506, 1014.5379, 1016.8979, 1019.2311, 1021.538, 1023.8188; 999.6579, 999.7009, 1002.0303, 1004.382, 1006.7084, 1009.0101, 1011.2874, 1013.5407, 1015.7703, 1017.9766, 1020.1599, 1022.3206; 998.1632, 998.2045, 1000.4375, 1002.6924, 1004.9239, 1007.1324, 1009.3183, 1011.4819, 1013.6236, 1015.7438, 1017.8428, 1019.921; 995.6057, 995.6458, 997.81864, 1000.0128, 1002.1841, 1004.3332, 1006.4603, 1008.566, 1010.6505, 1012.7144, 1014.758, 1016.7815; 992.1724, 992.2119, 994.35133, 996.5113, 998.6484, 1000.7633, 1002.8563, 1004.928, 1006.9788, 1009.009, 1011.0192, 1013.0097; 988.02, 988.0299, 990.15684, 992.3035, 994.4268, 996.5273, 998.6056, 1000.6622, 1002.6976, 1004.7123, 1006.7067, 1008.6813; 983.18, 983.1901, 985.3217, 987.4721, 989.5983, 991.7008, 993.7803, 995.8374, 997.8726, 999.8864, 1001.8795, 1003.8522; 977.75, 977.7583, 979.9094, 982.0783, 984.2216, 986.34, 988.4343, 990.505, 992.5529, 994.5786, 996.5825, 998.5654; 971.77, 971.7836, 973.96734, 976.1678, 978.3409, 980.4876, 982.6087, 984.7049, 986.7768, 988.8254, 990.8511, 992.8545; 965.26, 965.3023, 967.53107, 969.7753, 971.9901, 974.1764, 976.3354, 978.4676, 980.5741, 982.6556, 984.7129, 986.7465; 958.62, 958.6315, 960.627, 962.9267, 965.1944, 967.4314, 969.6387, 971.8173, 973.9681, 976.0921, 978.19, 980.2628] kg/m^3  rho_ref_3=998.21 kg/m^3  T_ref_3=293.16 K  p_ref_3=0.101325 MPa  beta_const_3=2.1791 GPa  alpha_const_3=2.0691e-4 1/K  rho_TLU_4=[999.84; 999.7; 998.2; 995.65; 992.21; 988.03; 983.19; 977.76; 971.78; 965.3; 958.8] kg/m^3  beta_const_4=2.1791 GPa  p_ref_4=0.101325 MPa  rho_ref_5=998.21 kg/m^3  T_ref_5=293.16 K  p_ref_5=0.101325 MPa  beta_const_5=2.1791 GPa  alpha_const_5=2.0691e-4 1/K  u_parameterization_2D=foundation.enum.u_parameterization_2D.u_cp  u_parameterization_1D=foundation.enum.u_parameterization_1D.u  u_TLU=[.0002, .0018, .086, .1588, .219, .267, .3034, .3288, .3436, .3483, .3435, .3294; 42.062, 42.06, 41.935, 41.804, 41.668, 41.527, 41.382, 41.233, 41.081, 40.924, 40.763, 40.599; 83.953, 83.948, 83.651, 83.349, 83.049, 82.749, 82.451, 82.153, 81.856, 81.56, 81.265, 80.971; 125.77, 125.76, 125.31, 124.86, 124.41, 123.97, 123.53, 123.1, 122.68, 122.25, 121.84, 121.42; 167.57, 167.56, 166.96, 166.37, 165.79, 165.21, 164.65, 164.09, 163.54, 163, 162.46, 161.94; 209.36, 209.36, 208.63, 207.9, 207.19, 206.48, 205.79, 205.11, 204.45, 203.79, 203.14, 202.5; 251.19, 251.19, 250.33, 249.47, 248.62, 247.79, 246.98, 246.18, 245.39, 244.62, 243.86, 243.12; 293.06, 293.06, 292.07, 291.07, 290.1, 289.14, 288.2, 287.28, 286.38, 285.49, 284.62, 283.77; 334.99, 334.99, 333.86, 332.73, 331.63, 330.54, 329.48, 328.44, 327.41, 326.41, 325.43, 324.46; 377, 377, 375.73, 374.46, 373.22, 372, 370.81, 369.64, 368.5, 367.38, 366.27, 365.19; 419.01, 419.01, 417.69, 416.27, 414.89, 413.54, 412.21, 410.91, 409.64, 408.4, 407.17, 405.98] kJ/kg  cp_TLU=[4.2199, 4.2194, 4.1957, 4.1726, 4.1508, 4.13, 4.1103, 4.0916, 4.0738, 4.0569, 4.0408, 4.0254; 4.1955, 4.1951, 4.1769, 4.1592, 4.1422, 4.1259, 4.1103, 4.0954, 4.0812, 4.0676, 4.0545, 4.0421; 4.1843, 4.184, 4.169, 4.1543, 4.1401, 4.1264, 4.1133, 4.1007, 4.0885, 4.0768, 4.0656, 4.0548; 4.1801, 4.1798, 4.1667, 4.1538, 4.1413, 4.1293, 4.1177, 4.1064, 4.0956, 4.0851, 4.075, 4.0653; 4.1796, 4.1794, 4.1675, 4.1558, 4.1444, 4.1334, 4.1227, 4.1123, 4.1023, 4.0926, 4.0832, 4.0741; 4.1813, 4.1813, 4.1702, 4.1592, 4.1484, 4.138, 4.1279, 4.1181, 4.1086, 4.0993, 4.0903, 4.0816; 4.185, 4.185, 4.1742, 4.1636, 4.1532, 4.1432, 4.1334, 4.1239, 4.1146, 4.1056, 4.0969, 4.0884; 4.1901, 4.1901, 4.1795, 4.169, 4.1588, 4.1489, 4.1393, 4.1299, 4.1207, 4.1118, 4.1032, 4.0947; 4.1968, 4.1968, 4.1862, 4.1757, 4.1655, 4.1555, 4.1458, 4.1364, 4.1273, 4.1183, 4.1096, 4.1012; 4.2052, 4.2052, 4.1944, 4.1837, 4.1733, 4.1632, 4.1534, 4.1438, 4.1345, 4.1255, 4.1166, 4.108; 4.2136, 4.2136, 4.2045, 4.1935, 4.1828, 4.1724, 4.1623, 4.1524, 4.1429, 4.1335, 4.1245, 4.1157] kJ/kg/K  u_TLU_2=[.0002, .0018, .086, .1588, .219, .267, .3034, .3288, .3436, .3483, .3435, .3294; 42.062, 42.06, 41.935, 41.804, 41.668, 41.527, 41.382, 41.233, 41.081, 40.924, 40.763, 40.599; 83.953, 83.948, 83.651, 83.349, 83.049, 82.749, 82.451, 82.153, 81.856, 81.56, 81.265, 80.971; 125.77, 125.76, 125.31, 124.86, 124.41, 123.97, 123.53, 123.1, 122.68, 122.25, 121.84, 121.42; 167.57, 167.56, 166.96, 166.37, 165.79, 165.21, 164.65, 164.09, 163.54, 163, 162.46, 161.94; 209.36, 209.36, 208.63, 207.9, 207.19, 206.48, 205.79, 205.11, 204.45, 203.79, 203.14, 202.5; 251.19, 251.19, 250.33, 249.47, 248.62, 247.79, 246.98, 246.18, 245.39, 244.62, 243.86, 243.12; 293.06, 293.06, 292.07, 291.07, 290.1, 289.14, 288.2, 287.28, 286.38, 285.49, 284.62, 283.77; 334.99, 334.99, 333.86, 332.73, 331.63, 330.54, 329.48, 328.44, 327.41, 326.41, 325.43, 324.46; 377, 377, 375.73, 374.46, 373.22, 372, 370.81, 369.64, 368.5, 367.38, 366.27, 365.19; 419.01, 419.01, 417.69, 416.27, 414.89, 413.54, 412.21, 410.91, 409.64, 408.4, 407.17, 405.98] kJ/kg  cp_TLU_3=[4.2199, 4.2194, 4.1957, 4.1726, 4.1508, 4.13, 4.1103, 4.0916, 4.0738, 4.0569, 4.0408, 4.0254; 4.1955, 4.1951, 4.1769, 4.1592, 4.1422, 4.1259, 4.1103, 4.0954, 4.0812, 4.0676, 4.0545, 4.0421; 4.1843, 4.184, 4.169, 4.1543, 4.1401, 4.1264, 4.1133, 4.1007, 4.0885, 4.0768, 4.0656, 4.0548; 4.1801, 4.1798, 4.1667, 4.1538, 4.1413, 4.1293, 4.1177, 4.1064, 4.0956, 4.0851, 4.075, 4.0653; 4.1796, 4.1794, 4.1675, 4.1558, 4.1444, 4.1334, 4.1227, 4.1123, 4.1023, 4.0926, 4.0832, 4.0741; 4.1813, 4.1813, 4.1702, 4.1592, 4.1484, 4.138, 4.1279, 4.1181, 4.1086, 4.0993, 4.0903, 4.0816; 4.185, 4.185, 4.1742, 4.1636, 4.1532, 4.1432, 4.1334, 4.1239, 4.1146, 4.1056, 4.0969, 4.0884; 4.1901, 4.1901, 4.1795, 4.169, 4.1588, 4.1489, 4.1393, 4.1299, 4.1207, 4.1118, 4.1032, 4.0947; 4.1968, 4.1968, 4.1862, 4.1757, 4.1655, 4.1555, 4.1458, 4.1364, 4.1273, 4.1183, 4.1096, 4.1012; 4.2052, 4.2052, 4.1944, 4.1837, 4.1733, 4.1632, 4.1534, 4.1438, 4.1345, 4.1255, 4.1166, 4.108; 4.2136, 4.2136, 4.2045, 4.1935, 4.1828, 4.1724, 4.1623, 4.1524, 4.1429, 4.1335, 4.1245, 4.1157] kJ/kg/K  u_TLU_4=[.0018; 42.06; 83.948; 125.76; 167.56; 209.36; 251.19; 293.06; 334.99; 377; 418.01] kJ/kg  cp_TLU_5=[4.2199; 4.1955; 4.1843; 4.1801; 4.1796; 4.1813; 4.185; 4.1901; 4.1968; 4.2052; 4.2136] kJ/kg/K  nu_TLU=[1.7917, 1.7914, 1.7763, 1.7615, 1.7473, 1.7338, 1.7208, 1.7085, 1.6967, 1.6854, 1.6747, 1.6645; 1.3061, 1.3059, 1.2986, 1.2914, 1.2845, 1.2779, 1.2716, 1.2656, 1.2598, 1.2543, 1.2491, 1.2441; 1.0032, 1.0032, .9995, .9959, .9924, .9891, .9859, .9829, .9801, .9774, .9748, .9724; .8006, .8005, .7987, .797, .7953, .7937, .7922, .7908, .7894, .7881, .787, .7859; .6577, .6577, .657, .6562, .6555, .6548, .6543, .6537, .6532, .6528, .6523, .652; .553, .553, .5529, .5527, .5526, .5525, .5524, .5524, .5524, .5524, .5524, .5525; .4739, .4739, .4741, .4743, .4745, .4747, .475, .4753, .4755, .4758, .4762, .4765; .4127, .4127, .4131, .4135, .4139, .4143, .4148, .4152, .4157, .4162, .4167, .4172; .3643, .3643, .3648, .3654, .3659, .3665, .367, .3676, .3682, .3688, .3694, .37; .3254, .3254, .3261, .3267, .3273, .328, .3286, .3293, .3299, .3306, .3312, .3319; .2866, .2866, .2945, .2952, .2959, .2965, .2972, .2979, .2986, .2993, .3, .3007] mm^2/s  nu_TLU_2=[1.7917; 1.3061; 1.0032; .8006; .6577; .553; .4739; .4127; .3643; .3254; .2866] mm^2/s  k_TLU=[561.04, 561.09, 563.8, 566.56, 569.32, 572.08, 574.82, 577.54, 580.24, 582.92, 585.57, 588.18; 580.02, 580.07, 582.45, 584.88, 587.32, 589.75, 592.18, 594.61, 597.02, 599.42, 601.8, 604.16; 598.44, 598.48, 600.73, 603.03, 605.33, 607.64, 609.94, 612.24, 614.54, 616.82, 619.1, 621.36; 615.48, 615.52, 617.73, 620, 622.26, 624.54, 626.81, 629.07, 631.34, 633.6, 635.85, 638.09; 630.6, 630.64, 632.87, 635.15, 637.44, 639.72, 642.01, 644.29, 646.57, 648.84, 651.11, 653.36; 643.61, 643.61, 645.88, 648.21, 650.53, 652.86, 655.18, 657.51, 659.82, 662.14, 664.44, 666.74; 654.39, 654.39, 656.73, 659.12, 661.5, 663.89, 666.27, 668.65, 671.02, 673.38, 675.74, 678.09; 663.13, 663.13, 665.54, 668, 670.46, 672.91, 675.36, 677.8, 680.24, 682.67, 685.09, 687.5; 670.02, 670.02, 672.51, 675.05, 677.59, 680.12, 682.64, 685.16, 687.67, 690.17, 692.66, 695.14; 675.27, 675.27, 677.85, 680.48, 683.11, 685.73, 688.34, 690.94, 693.53, 696.11, 698.68, 701.24; 680.52, 680.52, 681.77, 684.5, 687.22, 689.94, 692.64, 695.34, 698.02, 700.69, 703.35, 706] mW/m/K  k_TLU_2=[561.04; 580.02; 598.44; 615.48; 630.6; 643.61; 654.39; 663.13; 670.02; 675.27; 680.52] mW/m/K
      settings: SourceProductBaseCode=SS
  Thermal Liquid Settings (TL)1 : fl_lib/Thermal Liquid/Utilities/Thermal Liquid Settings (TL)  table_dimensions=foundation.enum.table_dimensions_TL.two_dimensional  T_TLU=[5 : 10 : 105]' degC  p_TLU=[0.01, 0.1, 5 : 5 : 50] MPa  p_atm=0.101325 MPa  pT_region_flag=foundation.enum.pT_region_TL.min_max  T_min=5 degC  T_max=105 degC  p_min=0.05 MPa  p_max=50 MPa  T_min_1D=273.16 K  T_max_1D=363.16 K  p_min_1D=0.05 MPa  p_max_1D=50 MPa  pT_validity_TLU=[1, 1, 1, 1, 1, 1, 1, 1, 1, 1, 1, 1; 1, 1, 1, 1, 1, 1, 1, 1, 1, 1, 1, 1; 1, 1, 1, 1, 1, 1, 1, 1, 1, 1, 1, 1; 1, 1, 1, 1, 1, 1, 1, 1, 1, 1, 1, 1; 1, 1, 1, 1, 1, 1, 1, 1, 1, 1, 1, 1; 0, 1, 1, 1, 1, 1, 1, 1, 1, 1, 1, 1; 0, 1, 1, 1, 1, 1, 1, 1, 1, 1, 1, 1; 0, 1, 1, 1, 1, 1, 1, 1, 1, 1, 1, 1; 0, 1, 1, 1, 1, 1, 1, 1, 1, 1, 1, 1; 0, 1, 1, 1, 1, 1, 1, 1, 1, 1, 1, 1; 0, 0, 1, 1, 1, 1, 1, 1, 1, 1, 1, 1]  rho_parameterization_2D=foundation.enum.rho_parameterization_2D.rho_beta_alpha  rho_parameterization_1D=foundation.enum.rho_parameterization_1D.rho_vector  rho_TLU=[999.7973, 999.8431, 1002.3216, 1004.8218, 1007.293, 1009.7358, 1012.1506, 1014.5379, 1016.8979, 1019.2311, 1021.538, 1023.8188; 999.6579, 999.7009, 1002.0303, 1004.382, 1006.7084, 1009.0101, 1011.2874, 1013.5407, 1015.7703, 1017.9766, 1020.1599, 1022.3206; 998.1632, 998.2045, 1000.4375, 1002.6924, 1004.9239, 1007.1324, 1009.3183, 1011.4819, 1013.6236, 1015.7438, 1017.8428, 1019.921; 995.6057, 995.6458, 997.81864, 1000.0128, 1002.1841, 1004.3332, 1006.4603, 1008.566, 1010.6505, 1012.7144, 1014.758, 1016.7815; 992.1724, 992.2119, 994.35133, 996.5113, 998.6484, 1000.7633, 1002.8563, 1004.928, 1006.9788, 1009.009, 1011.0192, 1013.0097; 988.02, 988.0299, 990.15684, 992.3035, 994.4268, 996.5273, 998.6056, 1000.6622, 1002.6976, 1004.7123, 1006.7067, 1008.6813; 983.18, 983.1901, 985.3217, 987.4721, 989.5983, 991.7008, 993.7803, 995.8374, 997.8726, 999.8864, 1001.8795, 1003.8522; 977.75, 977.7583, 979.9094, 982.0783, 984.2216, 986.34, 988.4343, 990.505, 992.5529, 994.5786, 996.5825, 998.5654; 971.77, 971.7836, 973.96734, 976.1678, 978.3409, 980.4876, 982.6087, 984.7049, 986.7768, 988.8254, 990.8511, 992.8545; 965.26, 965.3023, 967.53107, 969.7753, 971.9901, 974.1764, 976.3354, 978.4676, 980.5741, 982.6556, 984.7129, 986.7465; 958.62, 958.6315, 960.627, 962.9267, 965.1944, 967.4314, 969.6387, 971.8173, 973.9681, 976.0921, 978.19, 980.2628] kg/m^3  beta_TLU=[1.9649, 1.9654, 1.9929, 2.0213, 2.0499, 2.0787, 2.1078, 2.1372, 2.1668, 2.1966, 2.2268, 2.2572; 2.0913, 2.0918, 2.1191, 2.1471, 2.1752, 2.2036, 2.2322, 2.261, 2.2899, 2.3191, 2.3485, 2.3781; 2.1786, 2.1791, 2.2067, 2.235, 2.2634, 2.2919, 2.3206, 2.3494, 2.3784, 2.4075, 2.4367, 2.4661; 2.2332, 2.2337, 2.2619, 2.2908, 2.3197, 2.3487, 2.3778, 2.407, 2.4363, 2.4657, 2.4951, 2.5246; 2.26, 2.2605, 2.2895, 2.3191, 2.3487, 2.3784, 2.4081, 2.4378, 2.4675, 2.4973, 2.5272, 2.5571; 2.2638, 2.2638, 2.2936, 2.324, 2.3544, 2.3848, 2.4151, 2.4455, 2.4758, 2.5062, 2.5365, 2.5669; 2.2472, 2.2472, 2.2779, 2.3092, 2.3403, 2.3715, 2.4025, 2.4336, 2.4646, 2.4955, 2.5264, 2.5573; 2.214, 2.214, 2.2455, 2.2776, 2.3096, 2.3415, 2.3733, 2.405, 2.4367, 2.4683, 2.4998, 2.5313; 2.1668, 2.1668, 2.1992, 2.2321, 2.2649, 2.2976, 2.3301, 2.3626, 2.3949, 2.4272, 2.4593, 2.4914; 2.1081, 2.1081, 2.1413, 2.175, 2.2086, 2.2421, 2.2754, 2.3085, 2.3415, 2.3744, 2.4072, 2.4399; 2.0494, 2.0494, 2.0739, 2.1084, 2.1428, 2.177, 2.211, 2.2449, 2.2786, 2.3121, 2.3455, 2.3788] GPa  alpha_TLU=1e-4 * [-.679, -.676, -.49, -.307, -.13, .041, .206, .365, .519, .668, .811, .949; .878, .881, .998, 1.114, 1.227, 1.337, 1.445, 1.549, 1.651, 1.75, 1.846, 1.939; 2.068, 2.069, 2.141, 2.213, 2.283, 2.352, 2.42, 2.486, 2.551, 2.614, 2.676, 2.736; 3.034, 3.035, 3.074, 3.113, 3.152, 3.191, 3.229, 3.267, 3.305, 3.341, 3.377, 3.413; 3.855, 3.856, 3.87, 3.884, 3.899, 3.914, 3.93, 3.946, 3.961, 3.977, 3.993, 4.009; 4.578, 4.578, 4.572, 4.566, 4.562, 4.558, 4.555, 4.552, 4.55, 4.549, 4.548, 4.547; 5.233, 5.233, 5.209, 5.186, 5.165, 5.144, 5.125, 5.107, 5.09, 5.074, 5.059, 5.045; 5.84, 5.84, 5.801, 5.762, 5.725, 5.691, 5.657, 5.625, 5.595, 5.566, 5.538, 5.512; 6.414, 6.414, 6.36, 6.307, 6.256, 6.208, 6.161, 6.117, 6.074, 6.033, 5.994, 5.956; 6.967, 6.967, 6.898, 6.831, 6.766, 6.705, 6.646, 6.589, 6.535, 6.482, 6.432, 6.384; 7.519, 7.519, 7.423, 7.342, 7.264, 7.189, 7.118, 7.049, 6.983, 6.92, 6.859, 6.8] 1/K  rho_TLU_2=[999.7973, 999.8431, 1002.3216, 1004.8218, 1007.293, 1009.7358, 1012.1506, 1014.5379, 1016.8979, 1019.2311, 1021.538, 1023.8188; 999.6579, 999.7009, 1002.0303, 1004.382, 1006.7084, 1009.0101, 1011.2874, 1013.5407, 1015.7703, 1017.9766, 1020.1599, 1022.3206; 998.1632, 998.2045, 1000.4375, 1002.6924, 1004.9239, 1007.1324, 1009.3183, 1011.4819, 1013.6236, 1015.7438, 1017.8428, 1019.921; 995.6057, 995.6458, 997.81864, 1000.0128, 1002.1841, 1004.3332, 1006.4603, 1008.566, 1010.6505, 1012.7144, 1014.758, 1016.7815; 992.1724, 992.2119, 994.35133, 996.5113, 998.6484, 1000.7633, 1002.8563, 1004.928, 1006.9788, 1009.009, 1011.0192, 1013.0097; 988.02, 988.0299, 990.15684, 992.3035, 994.4268, 996.5273, 998.6056, 1000.6622, 1002.6976, 1004.7123, 1006.7067, 1008.6813; 983.18, 983.1901, 985.3217, 987.4721, 989.5983, 991.7008, 993.7803, 995.8374, 997.8726, 999.8864, 1001.8795, 1003.8522; 977.75, 977.7583, 979.9094, 982.0783, 984.2216, 986.34, 988.4343, 990.505, 992.5529, 994.5786, 996.5825, 998.5654; 971.77, 971.7836, 973.96734, 976.1678, 978.3409, 980.4876, 982.6087, 984.7049, 986.7768, 988.8254, 990.8511, 992.8545; 965.26, 965.3023, 967.53107, 969.7753, 971.9901, 974.1764, 976.3354, 978.4676, 980.5741, 982.6556, 984.7129, 986.7465; 958.62, 958.6315, 960.627, 962.9267, 965.1944, 967.4314, 969.6387, 971.8173, 973.9681, 976.0921, 978.19, 980.2628] kg/m^3  rho_ref_3=998.21 kg/m^3  T_ref_3=293.16 K  p_ref_3=0.101325 MPa  beta_const_3=2.1791 GPa  alpha_const_3=2.0691e-4 1/K  rho_TLU_4=[999.84; 999.7; 998.2; 995.65; 992.21; 988.03; 983.19; 977.76; 971.78; 965.3; 958.8] kg/m^3  beta_const_4=2.1791 GPa  p_ref_4=0.101325 MPa  rho_ref_5=998.21 kg/m^3  T_ref_5=293.16 K  p_ref_5=0.101325 MPa  beta_const_5=2.1791 GPa  alpha_const_5=2.0691e-4 1/K  u_parameterization_2D=foundation.enum.u_parameterization_2D.u_cp  u_parameterization_1D=foundation.enum.u_parameterization_1D.u  u_TLU=[.0002, .0018, .086, .1588, .219, .267, .3034, .3288, .3436, .3483, .3435, .3294; 42.062, 42.06, 41.935, 41.804, 41.668, 41.527, 41.382, 41.233, 41.081, 40.924, 40.763, 40.599; 83.953, 83.948, 83.651, 83.349, 83.049, 82.749, 82.451, 82.153, 81.856, 81.56, 81.265, 80.971; 125.77, 125.76, 125.31, 124.86, 124.41, 123.97, 123.53, 123.1, 122.68, 122.25, 121.84, 121.42; 167.57, 167.56, 166.96, 166.37, 165.79, 165.21, 164.65, 164.09, 163.54, 163, 162.46, 161.94; 209.36, 209.36, 208.63, 207.9, 207.19, 206.48, 205.79, 205.11, 204.45, 203.79, 203.14, 202.5; 251.19, 251.19, 250.33, 249.47, 248.62, 247.79, 246.98, 246.18, 245.39, 244.62, 243.86, 243.12; 293.06, 293.06, 292.07, 291.07, 290.1, 289.14, 288.2, 287.28, 286.38, 285.49, 284.62, 283.77; 334.99, 334.99, 333.86, 332.73, 331.63, 330.54, 329.48, 328.44, 327.41, 326.41, 325.43, 324.46; 377, 377, 375.73, 374.46, 373.22, 372, 370.81, 369.64, 368.5, 367.38, 366.27, 365.19; 419.01, 419.01, 417.69, 416.27, 414.89, 413.54, 412.21, 410.91, 409.64, 408.4, 407.17, 405.98] kJ/kg  cp_TLU=[4.2199, 4.2194, 4.1957, 4.1726, 4.1508, 4.13, 4.1103, 4.0916, 4.0738, 4.0569, 4.0408, 4.0254; 4.1955, 4.1951, 4.1769, 4.1592, 4.1422, 4.1259, 4.1103, 4.0954, 4.0812, 4.0676, 4.0545, 4.0421; 4.1843, 4.184, 4.169, 4.1543, 4.1401, 4.1264, 4.1133, 4.1007, 4.0885, 4.0768, 4.0656, 4.0548; 4.1801, 4.1798, 4.1667, 4.1538, 4.1413, 4.1293, 4.1177, 4.1064, 4.0956, 4.0851, 4.075, 4.0653; 4.1796, 4.1794, 4.1675, 4.1558, 4.1444, 4.1334, 4.1227, 4.1123, 4.1023, 4.0926, 4.0832, 4.0741; 4.1813, 4.1813, 4.1702, 4.1592, 4.1484, 4.138, 4.1279, 4.1181, 4.1086, 4.0993, 4.0903, 4.0816; 4.185, 4.185, 4.1742, 4.1636, 4.1532, 4.1432, 4.1334, 4.1239, 4.1146, 4.1056, 4.0969, 4.0884; 4.1901, 4.1901, 4.1795, 4.169, 4.1588, 4.1489, 4.1393, 4.1299, 4.1207, 4.1118, 4.1032, 4.0947; 4.1968, 4.1968, 4.1862, 4.1757, 4.1655, 4.1555, 4.1458, 4.1364, 4.1273, 4.1183, 4.1096, 4.1012; 4.2052, 4.2052, 4.1944, 4.1837, 4.1733, 4.1632, 4.1534, 4.1438, 4.1345, 4.1255, 4.1166, 4.108; 4.2136, 4.2136, 4.2045, 4.1935, 4.1828, 4.1724, 4.1623, 4.1524, 4.1429, 4.1335, 4.1245, 4.1157] kJ/kg/K  u_TLU_2=[.0002, .0018, .086, .1588, .219, .267, .3034, .3288, .3436, .3483, .3435, .3294; 42.062, 42.06, 41.935, 41.804, 41.668, 41.527, 41.382, 41.233, 41.081, 40.924, 40.763, 40.599; 83.953, 83.948, 83.651, 83.349, 83.049, 82.749, 82.451, 82.153, 81.856, 81.56, 81.265, 80.971; 125.77, 125.76, 125.31, 124.86, 124.41, 123.97, 123.53, 123.1, 122.68, 122.25, 121.84, 121.42; 167.57, 167.56, 166.96, 166.37, 165.79, 165.21, 164.65, 164.09, 163.54, 163, 162.46, 161.94; 209.36, 209.36, 208.63, 207.9, 207.19, 206.48, 205.79, 205.11, 204.45, 203.79, 203.14, 202.5; 251.19, 251.19, 250.33, 249.47, 248.62, 247.79, 246.98, 246.18, 245.39, 244.62, 243.86, 243.12; 293.06, 293.06, 292.07, 291.07, 290.1, 289.14, 288.2, 287.28, 286.38, 285.49, 284.62, 283.77; 334.99, 334.99, 333.86, 332.73, 331.63, 330.54, 329.48, 328.44, 327.41, 326.41, 325.43, 324.46; 377, 377, 375.73, 374.46, 373.22, 372, 370.81, 369.64, 368.5, 367.38, 366.27, 365.19; 419.01, 419.01, 417.69, 416.27, 414.89, 413.54, 412.21, 410.91, 409.64, 408.4, 407.17, 405.98] kJ/kg  cp_TLU_3=[4.2199, 4.2194, 4.1957, 4.1726, 4.1508, 4.13, 4.1103, 4.0916, 4.0738, 4.0569, 4.0408, 4.0254; 4.1955, 4.1951, 4.1769, 4.1592, 4.1422, 4.1259, 4.1103, 4.0954, 4.0812, 4.0676, 4.0545, 4.0421; 4.1843, 4.184, 4.169, 4.1543, 4.1401, 4.1264, 4.1133, 4.1007, 4.0885, 4.0768, 4.0656, 4.0548; 4.1801, 4.1798, 4.1667, 4.1538, 4.1413, 4.1293, 4.1177, 4.1064, 4.0956, 4.0851, 4.075, 4.0653; 4.1796, 4.1794, 4.1675, 4.1558, 4.1444, 4.1334, 4.1227, 4.1123, 4.1023, 4.0926, 4.0832, 4.0741; 4.1813, 4.1813, 4.1702, 4.1592, 4.1484, 4.138, 4.1279, 4.1181, 4.1086, 4.0993, 4.0903, 4.0816; 4.185, 4.185, 4.1742, 4.1636, 4.1532, 4.1432, 4.1334, 4.1239, 4.1146, 4.1056, 4.0969, 4.0884; 4.1901, 4.1901, 4.1795, 4.169, 4.1588, 4.1489, 4.1393, 4.1299, 4.1207, 4.1118, 4.1032, 4.0947; 4.1968, 4.1968, 4.1862, 4.1757, 4.1655, 4.1555, 4.1458, 4.1364, 4.1273, 4.1183, 4.1096, 4.1012; 4.2052, 4.2052, 4.1944, 4.1837, 4.1733, 4.1632, 4.1534, 4.1438, 4.1345, 4.1255, 4.1166, 4.108; 4.2136, 4.2136, 4.2045, 4.1935, 4.1828, 4.1724, 4.1623, 4.1524, 4.1429, 4.1335, 4.1245, 4.1157] kJ/kg/K  u_TLU_4=[.0018; 42.06; 83.948; 125.76; 167.56; 209.36; 251.19; 293.06; 334.99; 377; 418.01] kJ/kg  cp_TLU_5=[4.2199; 4.1955; 4.1843; 4.1801; 4.1796; 4.1813; 4.185; 4.1901; 4.1968; 4.2052; 4.2136] kJ/kg/K  nu_TLU=[1.7917, 1.7914, 1.7763, 1.7615, 1.7473, 1.7338, 1.7208, 1.7085, 1.6967, 1.6854, 1.6747, 1.6645; 1.3061, 1.3059, 1.2986, 1.2914, 1.2845, 1.2779, 1.2716, 1.2656, 1.2598, 1.2543, 1.2491, 1.2441; 1.0032, 1.0032, .9995, .9959, .9924, .9891, .9859, .9829, .9801, .9774, .9748, .9724; .8006, .8005, .7987, .797, .7953, .7937, .7922, .7908, .7894, .7881, .787, .7859; .6577, .6577, .657, .6562, .6555, .6548, .6543, .6537, .6532, .6528, .6523, .652; .553, .553, .5529, .5527, .5526, .5525, .5524, .5524, .5524, .5524, .5524, .5525; .4739, .4739, .4741, .4743, .4745, .4747, .475, .4753, .4755, .4758, .4762, .4765; .4127, .4127, .4131, .4135, .4139, .4143, .4148, .4152, .4157, .4162, .4167, .4172; .3643, .3643, .3648, .3654, .3659, .3665, .367, .3676, .3682, .3688, .3694, .37; .3254, .3254, .3261, .3267, .3273, .328, .3286, .3293, .3299, .3306, .3312, .3319; .2866, .2866, .2945, .2952, .2959, .2965, .2972, .2979, .2986, .2993, .3, .3007] mm^2/s  nu_TLU_2=[1.7917; 1.3061; 1.0032; .8006; .6577; .553; .4739; .4127; .3643; .3254; .2866] mm^2/s  k_TLU=[561.04, 561.09, 563.8, 566.56, 569.32, 572.08, 574.82, 577.54, 580.24, 582.92, 585.57, 588.18; 580.02, 580.07, 582.45, 584.88, 587.32, 589.75, 592.18, 594.61, 597.02, 599.42, 601.8, 604.16; 598.44, 598.48, 600.73, 603.03, 605.33, 607.64, 609.94, 612.24, 614.54, 616.82, 619.1, 621.36; 615.48, 615.52, 617.73, 620, 622.26, 624.54, 626.81, 629.07, 631.34, 633.6, 635.85, 638.09; 630.6, 630.64, 632.87, 635.15, 637.44, 639.72, 642.01, 644.29, 646.57, 648.84, 651.11, 653.36; 643.61, 643.61, 645.88, 648.21, 650.53, 652.86, 655.18, 657.51, 659.82, 662.14, 664.44, 666.74; 654.39, 654.39, 656.73, 659.12, 661.5, 663.89, 666.27, 668.65, 671.02, 673.38, 675.74, 678.09; 663.13, 663.13, 665.54, 668, 670.46, 672.91, 675.36, 677.8, 680.24, 682.67, 685.09, 687.5; 670.02, 670.02, 672.51, 675.05, 677.59, 680.12, 682.64, 685.16, 687.67, 690.17, 692.66, 695.14; 675.27, 675.27, 677.85, 680.48, 683.11, 685.73, 688.34, 690.94, 693.53, 696.11, 698.68, 701.24; 680.52, 680.52, 681.77, 684.5, 687.22, 689.94, 692.64, 695.34, 698.02, 700.69, 703.35, 706] mW/m/K  k_TLU_2=[561.04; 580.02; 598.44; 615.48; 630.6; 643.61; 654.39; 663.13; 670.02; 675.27; 680.52] mW/m/K
      settings: SourceProductBaseCode=SS
  Thermal Mass : fl_lib/Thermal/Thermal Elements/Thermal Mass  mass=3 kg  sp_heat=450 J/(K*kg)  T_specify=off  T_priority=High  T=300 K  T_nominal_specify=off  T_nominal_unit=K  T_nominal_value=1  Q_specify=off  Q_priority=None  Q=0 W  Q_nominal_specify=off  Q_nominal_unit=W  Q_nominal_value=1
  Thermal Reference : fl_lib/Thermal/Thermal Elements/Thermal Reference
  Transfer Fcn : TransferFcn  Denominator=[2 1]
  Unit Delay : UnitDelay  SampleTime=0.01  HasFrameUpgradeWarning=on
  Volumetric Flow Rate Sensor (TL) : fl_lib/Thermal Liquid/Sensors/Volumetric Flow Rate Sensor (TL)
      settings: SourceProductBaseCode=SS  InternalSimscapePortConfiguration="{\"Bottom\":[],\"Left\":[{\"id\":\"A\",\"label\":\"A\",\"type\":\"foundation.thermal_liquid.thermal_liquid\"}],\"Right\":[{\"id\":\"B\",\"label\":\"B\",\"type\":\"foundation.thermal_liquid.thermal_liquid\"},{\"id\":\"V\",\"label\":\"V\",\"type\":\"output\"}],\"Top\":[]}"
  Volumetric Flow Rate Sensor (TL)1 : fl_lib/Thermal Liquid/Sensors/Volumetric Flow Rate Sensor (TL)
      settings: SourceProductBaseCode=SS  InternalSimscapePortConfiguration="{\"Bottom\":[],\"Left\":[{\"id\":\"A\",\"label\":\"A\",\"type\":\"foundation.thermal_liquid.thermal_liquid\"}],\"Right\":[{\"id\":\"B\",\"label\":\"B\",\"type\":\"foundation.thermal_liquid.thermal_liquid\"},{\"id\":\"V\",\"label\":\"V\",\"type\":\"output\"}],\"Top\":[]}"
  Zero-Order Hold : ZeroOrderHold  SampleTime=0.01
  Zero-Order Hold1 : ZeroOrderHold  SampleTime=0.01
  Zero-Order Hold2 : ZeroOrderHold  SampleTime=0.01
  wires:
  Saturation3/1 -> Gain5/1
  Gain5/1 -> Simulink-PS Converter2/1
  [Cmd] -> Zero-Order Hold1/1
  Transfer Fcn/1 -> Saturation/1
  Saturation/1 -> Manual Switch1/1, [Cmd]  "BasicAnalogOutput"
  Add1/1 -> Gain2/1
  [T1] -> Add/1
  MATLAB Function/2(maxSlope) -> Display5/1
  PS-Simulink Converter8/1 -> Display3/1
  Gain2/1 -> Subtract2/1  "AvgPress"
  Discrete Transfer Fcn/1 -> Zero-Order Hold/1
  PS-Simulink Converter11/1 -> [P3]
  PID Controller/1 -> Product/2
  Pump Motor Input/1 -> Gain4/1
  Constant4/1 -> Subtract2/2
  [P3] -> Add1/3
  PS-Simulink Converter10/1 -> [P2]
  [P4] -> Add1/4
  Subtract2/1 -> Gain3/1
  Gain1/1 -> Saturation1/1
  PS-Simulink Converter9/1 -> [P1]
  Zero-Order Hold1/1 -> MATLAB Function/2(valveCmd)
  Product/1 -> Transfer Fcn/1
  [P2] -> Add1/2
  [P5] -> Add1/5
  Constant2/1 -> Simulink-PS Converter1/1
  Gain4/1 -> Saturation3/1
  Clock/1 -> Zero-Order Hold2/1
  [P1] -> Add1/1
  MATLAB Function/5(ssTime) -> Display6/1
  MATLAB Function/4(ssFlag) -> Terminator/1
  [T2] -> Add/2
  [T3] -> Add/3
  Subtract/1 -> Relay/1, PID Controller/1
  Gain3/1 -> Saturation2/1
  Constant5/1 -> MATLAB Function/4(Ts)
  Manual Voltage Control/1 -> Subsystem/1(In1)
  Zero-Order Hold/1 -> Scope1/1, MATLAB Function/1(T)
  PS-Simulink Converter7/1 -> [T5]
  Relay/1 -> Product/1
  PS-Simulink Converter3/1 -> Display2/1
  PS-Simulink Converter1/1 -> Display/1
  Constant1/1 -> Subtract1/2
  PS-Simulink Converter/1 -> [T3]
  Add/1 -> Gain/1
  PS-Simulink Converter12/1 -> [P4]
  PS-Simulink Converter2/1 -> Display1/1
  PS-Simulink Converter13/1 -> [P5]
  Saturation2/1 -> "Analog output v2 "/1
  Constant/1 -> Subtract/2
  PS-Simulink Converter6/1 -> [T4]
  Zero-Order Hold2/1 -> MATLAB Function/3(t)
  [Tavg] -> Discrete Transfer Fcn/1
  [T4] -> Add/4
  Saturation1/1 -> "Analog output v2 "/2
  PS-Simulink Converter5/1 -> [T2]
  MATLAB Function/1(dTdt) -> Scope/1
  Subtract1/1 -> Gain1/1
  PS-Simulink Converter4/1 -> [T1]
  [T5] -> Add/5
  Subsystem/1(Out1) -> Manual Switch/2
  Manual Switch/1 -> Simulink-PS Converter3/1
  Manual Switch1/1 -> Simulink-PS Converter/1
  Constant3/1 -> Saturation4/1
  Saturation4/1 -> Manual Switch1/2
  Subtract3/1 -> Relay1/1, Discrete PID Controller/1
  Saturation5/1 -> Display7/1, Manual Switch/1
  Constant6/1 -> Subtract3/1
  [Tavg] -> Subtract3/2  "AvgTemp"
  Gain/1 -> Unit Delay/1  "AvgTemp"
  Unit Delay/1 -> Subtract1/1, [Tavg], Subtract/1
  Relay1/1 -> Product1/1
  Discrete PID Controller/1 -> Product1/2
  Product1/1 -> Saturation5/1
  connections:
  Heat Exchanger (TL-TL)/LConn1 -- Pressure & Temperature Sensor (TL)1/LConn1 -- Reservoir (TL)4/LConn1 -- Thermal Liquid Settings (TL)1/RConn1
  Pipe (TL)/LConn1 -- Pressure & Temperature Sensor (TL)5/LConn1 -- Centrifugal Pump (TL)/LConn2
  Ideal Angular Velocity Source/RConn2 -- Mechanical Rotational Reference/LConn1 -- Centrifugal Pump (TL)/RConn2
  Pressure & Temperature Sensor (TL)4/LConn1 -- Pipe (TL)2/LConn1 -- Pipe (TL)1/RConn1
  Controlled Heat Flow Rate Source/LConn1 -- Conductive Heat Transfer6/LConn1 -- Pipe (TL)1/LConn2 -- Thermal Mass/LConn1
  Pressure & Temperature Sensor (TL)6/LConn1 -- Heat Exchanger (TL-TL)/RConn2 -- Thermal Liquid Settings (TL)/RConn1 -- Solver Configuration/RConn1 -- Centrifugal Pump (TL)/LConn1
  Ball Valve (TL)/LConn1 -- Pressure & Temperature Sensor (TL)3/LConn1 -- Pipe (TL)3/LConn1 -- Pipe (TL)2/RConn1
  Volumetric Flow Rate Sensor (TL)1/RConn1 -- Pressure & Temperature Sensor (TL)/LConn1 -- Pipe (TL)1/LConn1
  Flow Coefficient Parameterized Valve (TL)/LConn1 -- Pressure & Temperature Sensor (TL)2/LConn1 -- Heat Exchanger (TL-TL)/LConn2
  Flow Coefficient Parameterized Valve (TL)/RConn1 -- Volumetric Flow Rate Sensor (TL)/LConn1
  Conductive Heat Transfer1/RConn1 -- Convective Heat Transfer1/LConn1
  Thermal Reference/LConn1 -- Controlled Heat Flow Rate Source/RConn2
  Reservoir (TL)1/LConn1 -- Volumetric Flow Rate Sensor (TL)/RConn1
  Ideal Angular Velocity Source/LConn1 -- Centrifugal Pump (TL)/RConn1
  Pressure & Temperature Sensor (TL)1/RConn2 -- PS-Simulink Converter2/LConn1
  Volumetric Flow Rate Sensor (TL)1/RConn2 -- PS-Simulink Converter8/LConn1
  Absolute Reference (TL)4/LConn1 -- Pressure & Temperature Sensor (TL)4/RConn1
  Absolute Reference (TL)1/LConn1 -- Pressure & Temperature Sensor (TL)1/RConn1
  Temperature Source6/LConn1 -- Convective Heat Transfer6/RConn1
  Simulink-PS Converter1/RConn1 -- Ball Valve (TL)/LConn2
  Pressure & Temperature Sensor (TL)5/RConn2 -- PS-Simulink Converter12/LConn1
  Absolute Reference (TL)5/LConn1 -- Pressure & Temperature Sensor (TL)5/RConn1
  PS-Simulink Converter/LConn1 -- Pressure & Temperature Sensor (TL)/RConn3
  Absolute Reference (TL)2/LConn1 -- Pressure & Temperature Sensor (TL)2/RConn1
  Temperature Source1/LConn1 -- Convective Heat Transfer1/RConn1
  PS-Simulink Converter9/LConn1 -- Pressure & Temperature Sensor (TL)3/RConn2
  Pressure & Temperature Sensor (TL)6/RConn2 -- PS-Simulink Converter13/LConn1
  Absolute Reference (TL)6/LConn1 -- Pressure & Temperature Sensor (TL)6/RConn1
  Pipe (TL)3/LConn2 -- Conductive Heat Transfer2/LConn1
  Absolute Reference (TL)/LConn1 -- Pressure & Temperature Sensor (TL)/RConn1
  Volumetric Flow Rate Sensor (TL)/RConn2 -- PS-Simulink Converter1/LConn1
  Conductive Heat Transfer2/RConn1 -- Convective Heat Transfer2/LConn1
  Conductive Heat Transfer/RConn1 -- Convective Heat Transfer/LConn1
  Pipe (TL)3/RConn1 -- Heat Exchanger (TL-TL)/RConn1
  Volumetric Flow Rate Sensor (TL)1/LConn1 -- Pipe (TL)/RConn1
  Conductive Heat Transfer6/RConn1 -- Convective Heat Transfer6/LConn1
  Temperature Source2/LConn1 -- Convective Heat Transfer2/RConn1
  Pressure & Temperature Sensor (TL)/RConn2 -- PS-Simulink Converter11/LConn1
  Pipe (TL)2/LConn2 -- Conductive Heat Transfer1/LConn1
  Flow Coefficient Parameterized Valve (TL)/LConn2 -- Simulink-PS Converter/RConn1
  Reservoir (TL)2/LConn1 -- Ball Valve (TL)/RConn1
  Pipe (TL)/LConn2 -- Conductive Heat Transfer/LConn1
  PS-Simulink Converter5/LConn1 -- Pressure & Temperature Sensor (TL)4/RConn3
  Temperature Source/LConn1 -- Convective Heat Transfer/RConn1
  Absolute Reference (TL)3/LConn1 -- Pressure & Temperature Sensor (TL)3/RConn1
  PS-Simulink Converter10/LConn1 -- Pressure & Temperature Sensor (TL)4/RConn2
  Simulink-PS Converter2/RConn1 -- Ideal Angular Velocity Source/RConn1
  PS-Simulink Converter4/LConn1 -- Pressure & Temperature Sensor (TL)3/RConn3
  Pressure & Temperature Sensor (TL)2/RConn2 -- PS-Simulink Converter3/LConn1
  PS-Simulink Converter7/LConn1 -- Pressure & Temperature Sensor (TL)6/RConn3
  PS-Simulink Converter6/LConn1 -- Pressure & Temperature Sensor (TL)5/RConn3
  Controlled Heat Flow Rate Source/RConn1 -- Simulink-PS Converter3/RConn1
